simulink model "VIRTUAL_self_driving_stack_autoLocalize_v2"  (R2026a)
settings: Solver=ode1  StopTime=inf  FixedStep=1/500  EnableMultiTasking=on
values from neighbouring files (symbols this model uses):
  path_x4 = [-0.614 -0.604 -0.594 -0.584 -0.574 -0.564 -0.554 -0.544 -0.534 -0.524 -0.514 -0.504 ... (1761 elements, 1761x1)]    [SDCS_Paths_7.mat]
  path_y4 = [-1.0887 -1.0887 -1.0887 -1.0887 -1.0887 -1.0887 -1.0887 -1.0887 -1.0887 -1.0887 -1.0887 -1.0887 ... (1761 elements, 1761x1)]    [SDCS_Paths_7.mat]
undefined symbols (not defined in the file or in its folder): AAAF5050, CSI_Sample_Time, DiscIntNeverNeededParam, gcbh, height, HIL, ImageDisplay_Sample_Time, Initialization_Time, JPEG, K12, left, LiDAR_Sample_Time, MC, qc_get_step_size, RealSense_Sample_Time, top, video_display_show, width
libraries: quarc_library x67, simulink x5, visionconversions x1, visiontransforms x1, sl_discontinuities x1
(part 3 of 3)

== system VIRTUAL_self_driving_stack_autoLocalize_v2/rateTimingPlots/monitorTiming5 ==
  note: moniorTiming Module:
      |
      | This subsystem outputs the sample time and computation time of the model.
      |
      | Outputs:
      | sampleTime (s) n/a : Sample time (unfiltered and filtered) in seconds.
      | computationTime (s) n/a : Computation time (unfiltered and filtered) in seconds.
      |
      | Usage:
      | Compare the Sample Time (s) output to a constant (qc_get_step_size) to monitor whether or not the desired sample time is being achieved. The Computation Time (s) values should be lower than the corresponding sample time value to ensure that the solver has enough time per time step.
  note: Timing Performance
  Computation Time : quarc_library/Sources/Time/Computation Time  sample_time=LiDAR_Sample_Time  use_model=on  use_cpu_time=off
  Constant : Constant  Value=LiDAR_Sample_Time  SampleTime=-1
  Mux : Mux  Inputs=3
  Sample Time : quarc_library/Sources/Time/Sample Time  Priority=-99  sample_time=LiDAR_Sample_Time
  Timing (s) : Outport  VectorParamsAs1DForOutWhenUnconnected=off
  wires:
  Constant/1 -> Mux/2
  Sample Time/1 -> Mux/1
  Mux/1 -> Timing (s)/1
  Computation Time/1 -> Mux/3

== system VIRTUAL_self_driving_stack_autoLocalize_v2/rateTimingPlots/monitorTiming7 ==
  note: Timing Performance
  note: moniorTiming Module:
      |
      | This subsystem outputs the sample time and computation time of the model.
      |
      | Outputs:
      | sampleTime (s) n/a : Sample time (unfiltered and filtered) in seconds.
      | computationTime (s) n/a : Computation time (unfiltered and filtered) in seconds.
      |
      | Usage:
      | Compare the Sample Time (s) output to a constant (qc_get_step_size) to monitor whether or not the desired sample time is being achieved. The Computation Time (s) values should be lower than the corresponding sample time value to ensure that the solver has enough time per time step.
  Computation Time : quarc_library/Sources/Time/Computation Time  sample_time=1  use_model=on  use_cpu_time=off
  Constant : Constant  SampleTime=-1
  Mux : Mux  Inputs=3
  Sample Time : quarc_library/Sources/Time/Sample Time  Priority=-99  sample_time=1
  Timing (s) : Outport  VectorParamsAs1DForOutWhenUnconnected=off
  wires:
  Computation Time/1 -> Mux/3
  Mux/1 -> Timing (s)/1
  Sample Time/1 -> Mux/1
  Constant/1 -> Mux/2

== system VIRTUAL_self_driving_stack_autoLocalize_v2/readQCarDAC/counts to meters ==
  note: Estimate car speed from motor encoder counts rate
  note: v = 2*pi*r * omega (if omega is in rot/s)
      | v = r * omega (if omega is in rad/s)
      | r = 0.0342 m
  note: (Diff. pinion*pinion)/(Spur*Diff. spur)
  note: speedEstimation Module:
      |
      | This subsystem converts the motor speed measurements in counts/s to a useful longitudinal car speed in m/s.
      |
      | Inputs:
      | motorSpeed (counts/s) n/a : Drive motor speed measured using an encoder
      |
      | Outputs:
      | longitudinalCarSpeed (m/s) n/a : The platform's longitudinal speed (along the front-rear axis direction)
  motorSpeed (counts/s) : Inport
  counts to rotations : Gain  Gain=1/720/4
  gear ratios : Gain  Gain=(13*19)/(70*37)
  rot/s to rad/s : Gain  Gain=2*pi
  wheel radius : Gain  Gain=0.0342
  longitudinalCarSpeed (m/s) : Outport  VectorParamsAs1DForOutWhenUnconnected=off
  wires:
  motorSpeed (counts/s)/1 -> counts to rotations/1
  rot/s to rad/s/1 -> wheel radius/1  "wheel speed (rad/s)"
  counts to rotations/1 -> gear ratios/1  "motor speed (rot/s)"
  wheel radius/1 -> longitudinalCarSpeed (m/s)/1  "wheel speed (m/s)"
  gear ratios/1 -> rot/s to rad/s/1  "shaft speed (rots/s)"

== system VIRTUAL_self_driving_stack_autoLocalize_v2/readQCarDAC/counts//s to m//s ==
  note: speedEstimation Module:
      |
      | This subsystem converts the motor speed measurements in counts/s to a useful longitudinal car speed in m/s.
      |
      | Inputs:
      | motorSpeed (counts/s) n/a : Drive motor speed measured using an encoder
      |
      | Outputs:
      | longitudinalCarSpeed (m/s) n/a : The platform's longitudinal speed (along the front-rear axis direction)
  note: (Diff. pinion*pinion)/(Spur*Diff. spur)
  note: v = 2*pi*r * omega (if omega is in rot/s)
      | v = r * omega (if omega is in rad/s)
      | r = 0.0342 m
  note: Estimate car speed from motor encoder counts rate
  motorSpeed (counts/s) : Inport
  counts to rotations : Gain  Gain=1/720/4
  gear ratios : Gain  Gain=(13*19)/(70*37)
  rot/s to rad/s : Gain  Gain=2*pi
  wheel radius : Gain  Gain=0.0342
  longitudinalCarSpeed (m/s) : Outport  VectorParamsAs1DForOutWhenUnconnected=off
  wires:
  gear ratios/1 -> rot/s to rad/s/1  "shaft speed (rots/s)"
  wheel radius/1 -> longitudinalCarSpeed (m/s)/1  "wheel speed (m/s)"
  counts to rotations/1 -> gear ratios/1  "motor speed (rot/s)"
  rot/s to rad/s/1 -> wheel radius/1  "wheel speed (rad/s)"
  motorSpeed (counts/s)/1 -> counts to rotations/1

== system VIRTUAL_self_driving_stack_autoLocalize_v2/readQCarDAC/powerConsumptionMonitor ==
  note: Battery percentage calculation
  note: P = VI
  note: Electrical
      | power
      | consumed
  note: Power Monitoring Module:
      |
      | This subsystem monitors power consumption and provides a percentage battery remaining indicator.
      |
      | Inputs:
      | motorCurrent (A) n/a : Motor current being pulled by the main drive motor
      | batteryVoltage (V) {0, 12.6} : Current battery voltage reading
      |
      | Outputs:
      | motorPowerConsumption (W) n/a : Current power in Watts being pulled by the main drive motor
      | batteryLevel (%) {0,1} : Percentage battery level remaining
      |
      | Usage:
      | This is based on a maximum 3S battery voltage of 12.6 V (4.2V per cell) and minimum of 10.5 V (3.5V per cell)
  motorCurrent (A) [1] : Inport
  batteryVoltage (V) [1] : Inport  Port=2
  Divide : Product  Inputs=*/
  Gain : Gain  Gain=100
  Product : Product
  Subtract : Sum  Inputs=+-
  Subtract1 : Sum  Inputs=+-
  max voltage : Constant  Value=12.6
  min voltage : Constant  Value=10.5
  motorPowerConsumption (W) [1] : Outport  VectorParamsAs1DForOutWhenUnconnected=off
  batteryLevel (%) [1] : Outport  Port=2  VectorParamsAs1DForOutWhenUnconnected=off
  wires:
  Divide/1 -> Gain/1
  Subtract1/1 -> Divide/2
  Gain/1 -> batteryLevel (%) [1]/1
  Product/1 -> motorPowerConsumption (W) [1]/1
  min voltage/1 -> Subtract/2, Subtract1/2
  motorCurrent (A) [1]/1 -> Product/1
  max voltage/1 -> Subtract1/1
  Subtract/1 -> Divide/1
  batteryVoltage (V) [1]/1 -> Subtract/1, Product/2

== system VIRTUAL_self_driving_stack_autoLocalize_v2/speedController/realsenseObstacleDetectionSpeedAdjust ==
  obstacleDistance [1] (m) : Inport
  desiredSpeed [1] (m/s) : Inport  Port=2
  Constant : Constant  Value=0.375
  Constant2 : Constant  Value=0.6
  MATLAB Function : MATLAB Function  TreatAsAtomicUnit=on
  objectDetectionAdjustedSpeed [1] (m/s) : Outport  VectorParamsAs1DForOutWhenUnconnected=off
  wires:
  Constant2/1 -> MATLAB Function/3(nominal_tracking_distance)  "nominal tracking distance (m)"
  Constant/1 -> MATLAB Function/2(stop_distance)  "stop distance (m)"
  obstacleDistance [1] (m)/1 -> MATLAB Function/1(obstacle_distance)
  MATLAB Function/1(speed_cmd) -> objectDetectionAdjustedSpeed [1] (m/s)/1
  desiredSpeed [1] (m/s)/1 -> MATLAB Function/4(nominal_speed)

== system VIRTUAL_self_driving_stack_autoLocalize_v2/speedController/speedController ==
  note: Feedforward
  note: Feedback
  arm [1] (bool) : Inport
  desiredSpeed (m/s) : Inport  Port=2
  currentSpeed (m/s) : Inport  Port=3
  Add : Sum
  Add1 : Sum
  Compare To Zero : simulink/Logic and Bit Operations/Compare To Zero  relop===  OutDataTypeStr=boolean
  Integrator1 : Integrator  ExternalReset=either  LimitOutput=on  UpperSaturationLimit=0.4  LowerSaturationLimit=-0.4
  Kff (% / m/s) : Gain  Gain=0.1
  "Ki (% / m) " : Gain
  Kp (% / m/s) : Gain  Gain=.3
  Multiply : Product
  Multiply1 : Product
  Multiply2 : Product
  Speed_Tracking : Scope  NumInputPorts=2
  Sum : Sum  Inputs=|+-
  command saturation : Saturate  UpperLimit=5  LowerLimit=-5
  throttleCmd (%) : Outport  VectorParamsAs1DForOutWhenUnconnected=off
  wires:
  command saturation/1 -> Multiply1/1  "desired"
  arm [1] (bool)/1 -> Multiply2/2, Multiply1/2, Multiply/2
  currentSpeed (m/s)/1 -> Multiply/1  "meas"
  Multiply/1 -> Sum/2, Speed_Tracking/2  "measured"
  Add/1 -> Add1/2
  Add1/1 -> Multiply2/1  "%"
  Multiply1/1 -> Compare To Zero/1, Sum/1, Kff (% / m/s)/1, Speed_Tracking/1  "desired"
  Integrator1/1 -> Add/2
  Kp (% / m/s)/1 -> Add/1
  Compare To Zero/1 -> Integrator1/2
  Kff (% / m/s)/1 -> Add1/1
  Sum/1 -> "Ki (% / m) "/1, Kp (% / m/s)/1
  "Ki (% / m) "/1 -> Integrator1/1
  Multiply2/1 -> throttleCmd (%)/1  "pwm duty cycle"
  desiredSpeed (m/s)/1 -> command saturation/1

== system VIRTUAL_self_driving_stack_autoLocalize_v2/speedController/stopSignDetectionSpeedAdjust ==
  stopSignDetection : Inport
  speedIn : Inport  Port=2
  Constant : Constant  Value=0
  Display : Display
  Display1 : Display
  Elapsed : Scope
      settings: ActiveDisplayYMinimum=-1  ActiveDisplayYMaximum=1
  Less Than Threshold : Subsystem
  NOT : Logic  Operator=NOT  IconShape=distinctive  AllPortsSameDT=off  OutDataTypeStr=boolean
  OR : Logic  Operator=OR  IconShape=distinctive  AllPortsSameDT=off  OutDataTypeStr=boolean
  Switch : Switch  Criteria=u2 > Threshold  SaturateOnIntegerOverflow=off  InputSameDT=off
  Switch1 : Switch  Criteria=u2 > Threshold  SaturateOnIntegerOverflow=off  InputSameDT=off
  time elspsed or no stop sign : Display
  time within stop sign : Constant  Value=2
  speedOut : Outport  VectorParamsAs1DForOutWhenUnconnected=off
  wires:
  stopSignDetection/1 -> NOT/1, Display1/1, Switch/2, Less Than Threshold/1(signal)
  time within stop sign/1 -> Less Than Threshold/2(Duration Threshold)
  Constant/1 -> Switch/1
  speedIn/1 -> Switch1/1, Switch/3
  Less Than Threshold/1(elapsed) -> OR/2, Elapsed/1
  NOT/1 -> OR/1
  OR/1 -> Switch1/2, time elspsed or no stop sign/1
  Switch/1 -> Switch1/3
  Switch1/1 -> Display/1, speedOut/1

== system VIRTUAL_self_driving_stack_autoLocalize_v2/speedController/turnSpeedHandler ==
  speedCmd [1] (m/s) : Inport
  steeringCmd [1] (rad) : Inport  Port=2
  Cos ^ (attentuation) : Inport  Port=3
  Cos : Trigonometry  Operator=cos
  Product : Product
  Speed Comparison : Scope  NumInputPorts=2
  Square : Math  Operator=pow  SignedPower=on
  attenuationLimits : Saturate  UpperLimit=1  LowerLimit=.3
  attenuatedSpeedCmd [1] (m/s) : Outport  VectorParamsAs1DForOutWhenUnconnected=off
  wires:
  Cos/1 -> Square/1
  attenuationLimits/1 -> Product/2
  speedCmd [1] (m/s)/1 -> Product/1, Speed Comparison/1  "Input Speed"
  Cos ^ (attentuation)/1 -> Square/2
  Square/1 -> attenuationLimits/1
  Product/1 -> attenuatedSpeedCmd [1] (m/s)/1, Speed Comparison/2
  steeringCmd [1] (rad)/1 -> Cos/1  "input steering"

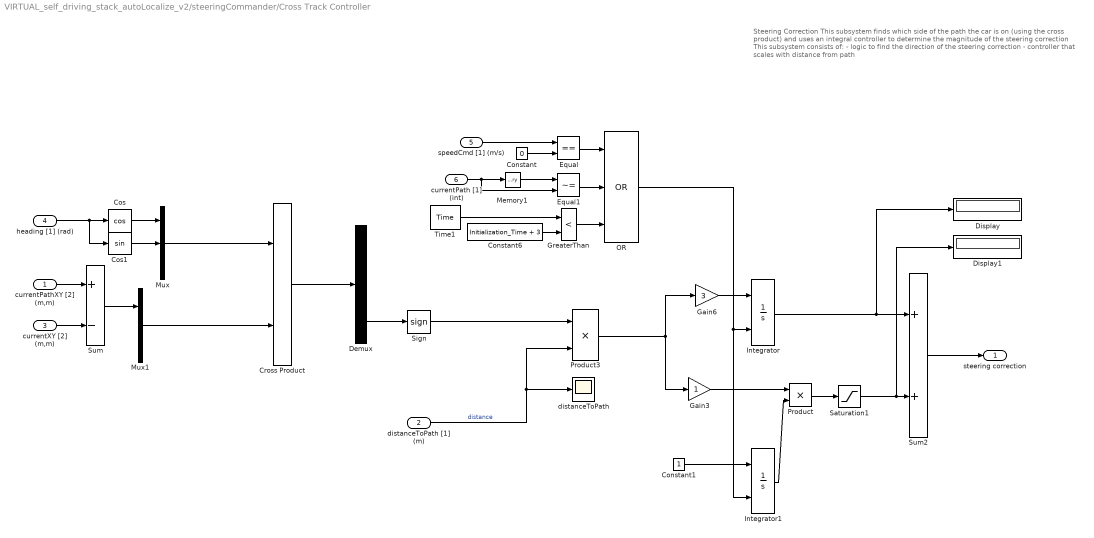
== system VIRTUAL_self_driving_stack_autoLocalize_v2/steeringCommander/Cross Track Controller ==
  note: Steering Correction
      |
      | This subsystem finds which side of the path the car is on (using the cross product) and uses an integral controller to determine the magnitude of the steering correction
      |
      | This subsystem consists of:
      |
      | - logic to find the direction of the steering correction
      | - controller that scales with distance from path
  currentPathXY [2] (m,m) : Inport
  distanceToPath [1] (m) : Inport  Port=2
  currentXY [2] (m,m) : Inport  Port=3
  heading [1] (rad) : Inport  Port=4
  speedCmd [1] (m/s) : Inport  Port=5
  currentPath [1] (int) : Inport  Port=6
  Constant : Constant  Value=0
  Constant1 : Constant
  Constant6 : Constant  Value=Initialization_Time + 3
  Cos : Trigonometry  Operator=cos
  Cos1 : Trigonometry
  Cross Product : quarc_library/Math Operations/Vectors/Cross Product
      settings: SourceProductName=QUARC Targets
  Demux : Demux  Outputs=3
  Display : Display
  Display1 : Display
  Equal : RelationalOperator  Operator===  OutDataTypeStr=boolean  RndMeth=Simplest  InputSameDT=off
  Equal1 : RelationalOperator  Operator=~=  OutDataTypeStr=boolean  RndMeth=Simplest  InputSameDT=off
  Gain3 : Gain
  Gain6 : Gain  Gain=3
  GreaterThan : RelationalOperator  Operator=<  OutDataTypeStr=boolean  RndMeth=Simplest  InputSameDT=off
  Integrator : Integrator  ExternalReset=level  LimitOutput=on  UpperSaturationLimit=.2  LowerSaturationLimit=-.2
  Integrator1 : Integrator  ExternalReset=level  LimitOutput=on  UpperSaturationLimit=1  LowerSaturationLimit=0
  Memory1 : Memory  InitialCondition=6  InheritSampleTime=on  LinearizeMemory=on  LinearizeAsDelay=on
  Mux : Mux  Inputs=3
  Mux1 : Mux  Inputs=2
  OR : Logic  Operator=OR  Inputs=3  IconShape=distinctive  AllPortsSameDT=off  OutDataTypeStr=boolean
  Product : Product
  Product3 : Product
  Saturation1 : Saturate  UpperLimit=.2  LowerLimit=-.2
  Sign : Signum
  Sum : Sum  Inputs=+-
  Sum2 : Sum
  Time1 : quarc_library/Sources/Time/Time  time_source=Wall clock  sample_time=qc_get_step_size
  distanceToPath : Scope
  steering correction : Outport
  wires:
  heading [1] (rad)/1 -> Cos1/1, Cos/1
  Cos/1 -> Mux/1
  Cos1/1 -> Mux/2
  currentXY [2] (m,m)/1 -> Sum/2
  currentPathXY [2] (m,m)/1 -> Sum/1
  Sum/1 -> Mux1/1
  Mux1/1 -> Cross Product/2
  Mux/1 -> Cross Product/1
  Cross Product/1 -> Demux/1
  Demux/3 -> Sign/1
  Sign/1 -> Product3/1
  Gain6/1 -> Integrator/1
  Product3/1 -> Gain3/1, Gain6/1
  Integrator/1 -> Display/1, Sum2/1
  Saturation1/1 -> Display1/1, Sum2/2
  distanceToPath [1] (m)/1 -> Product3/2, distanceToPath/1  "distance"
  Sum2/1 -> steering correction/1
  speedCmd [1] (m/s)/1 -> Equal/1
  Constant/1 -> Equal/2
  currentPath [1] (int)/1 -> Equal1/2, Memory1/1
  Memory1/1 -> Equal1/1
  Equal1/1 -> OR/2
  Equal/1 -> OR/1
  OR/1 -> Integrator1/2, Integrator/2
  Constant1/1 -> Integrator1/1
  Product/1 -> Saturation1/1
  Gain3/1 -> Product/1
  Integrator1/1 -> Product/2
  Time1/1 -> GreaterThan/1
  Constant6/1 -> GreaterThan/2
  GreaterThan/1 -> OR/3

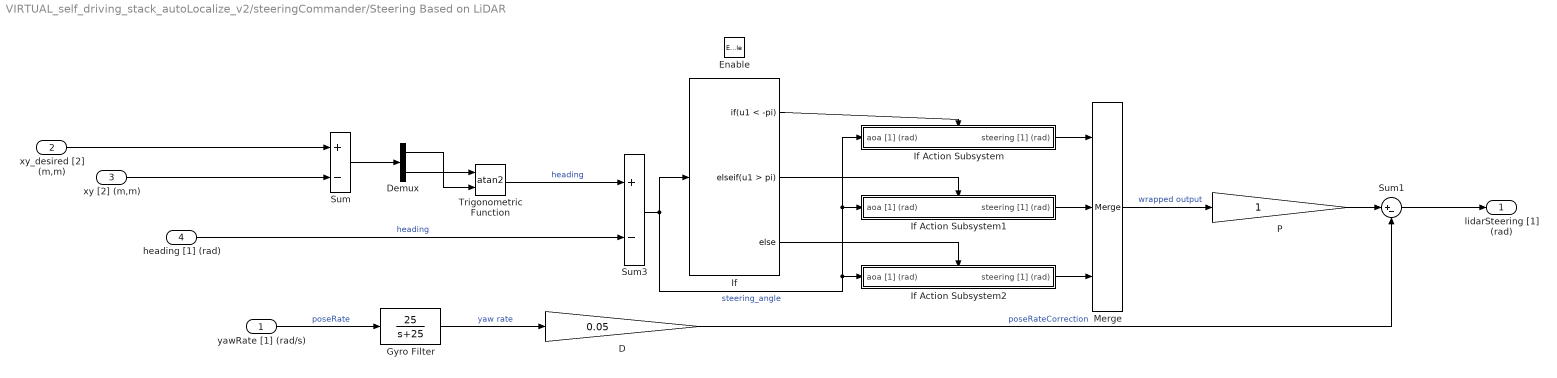
== system VIRTUAL_self_driving_stack_autoLocalize_v2/steeringCommander/Steering Based on LiDAR ==
  yawRate [1] (rad/s) : Inport
  xy_desired [2] (m,m) : Inport  Port=2
  xy [2] (m,m) : Inport  Port=3
  heading [1] (rad) : Inport  Port=4
  Enable : EnablePort  PropagateVarSize=During execution
  D : Gain  Gain=0.05
  Demux : Demux  Outputs=2
  Gyro Filter : TransferFcn  Numerator=[25]  Denominator=[1 25]
  If : If  IfExpression=u1 < -pi  ElseIfExpressions=u1 > pi
  If Action Subsystem : Subsystem  TreatAsAtomicUnit=on
  If Action Subsystem1 : Subsystem  TreatAsAtomicUnit=on
  If Action Subsystem2 : Subsystem  TreatAsAtomicUnit=on
  Merge : Merge  Inputs=3
  P : Gain
  Sum : Sum  Inputs=+-
  Sum1 : Sum  Inputs=|+-
  Sum3 : Sum  Inputs=+-
  Trigonometric Function : Trigonometry  Operator=atan2
  lidarSteering [1] (rad) : Outport
  wires:
  If/1 -> If Action Subsystem/Action
  If/2 -> If Action Subsystem1/Action
  If/3 -> If Action Subsystem2/Action
  Sum3/1 -> If Action Subsystem1/1(aoa [1] (rad)), If Action Subsystem/1(aoa [1] (rad)), If Action Subsystem2/1(aoa [1] (rad)), If/1  "steering_angle"
  If Action Subsystem/1(steering [1] (rad)) -> Merge/1
  If Action Subsystem1/1(steering [1] (rad)) -> Merge/2
  If Action Subsystem2/1(steering [1] (rad)) -> Merge/3
  Demux/1 -> Trigonometric Function/2
  xy [2] (m,m)/1 -> Sum/2
  xy_desired [2] (m,m)/1 -> Sum/1
  heading [1] (rad)/1 -> Sum3/2  "heading"
  Sum/1 -> Demux/1
  Demux/2 -> Trigonometric Function/1
  Merge/1 -> P/1  "wrapped output"
  D/1 -> Sum1/2  "poseRateCorrection"
  Sum1/1 -> lidarSteering [1] (rad)/1
  P/1 -> Sum1/1
  Trigonometric Function/1 -> Sum3/1  "heading"
  yawRate [1] (rad/s)/1 -> Gyro Filter/1  "poseRate"
  Gyro Filter/1 -> D/1  "yaw rate"

== system VIRTUAL_self_driving_stack_autoLocalize_v2/HSVStopSignDetection/findStopSignDistance/Depth Image (m) ==
  In1 : Inport
  Channel : quarc_library/Signal Routing/Channel  channel=0  buffer_size=1
  Image Compress : quarc_library/Image Processing/Generic/Image Compress  algorithm=JPEG  source=Internal dialog parameter  quality=quality  output_dim=-1
  Video Display : quarc_library/Multimedia/Video Display  Tag=VIRTUAL_self_driving_stack_autoLocalize_v2/HSVStopSignDetection/findStopSignDistance/Depth Image (m)/Video Display  sample_time=sample_time  use_hardware=on
  wires:
  Image Compress/1 -> Channel/1
  In1/1 -> Image Compress/1
  Channel/1 -> Video Display/1

== system VIRTUAL_self_driving_stack_autoLocalize_v2/HSVStopSignDetection/findStopSignLocation/Binary showing blob found ==
  In1 : Inport
  Channel : quarc_library/Signal Routing/Channel  channel=1  buffer_size=1
  Image Compress : quarc_library/Image Processing/Generic/Image Compress  algorithm=JPEG  source=Internal dialog parameter  quality=quality  output_dim=-1
  Video Display : quarc_library/Multimedia/Video Display  Tag=<binary blob, 124 chars, not shown>  sample_time=sample_time  use_hardware=on
  wires:
  Image Compress/1 -> Channel/1
  In1/1 -> Image Compress/1
  Channel/1 -> Video Display/1

== system VIRTUAL_self_driving_stack_autoLocalize_v2/HSVStopSignDetection/findStopSignLocation/Raw RGB ==
  In1 : Inport
  Channel : quarc_library/Signal Routing/Channel  channel=2  buffer_size=1
  Image Compress : quarc_library/Image Processing/Generic/Image Compress  algorithm=JPEG  source=Internal dialog parameter  quality=quality  output_dim=-1
  Video Display : quarc_library/Multimedia/Video Display  Tag=VIRTUAL_self_driving_stack_autoLocalize_v2/HSVStopSignDetection/findStopSignLocation/Raw RGB/Video Display  sample_time=sample_time  use_hardware=on
  wires:
  Image Compress/1 -> Channel/1
  In1/1 -> Image Compress/1
  Channel/1 -> Video Display/1

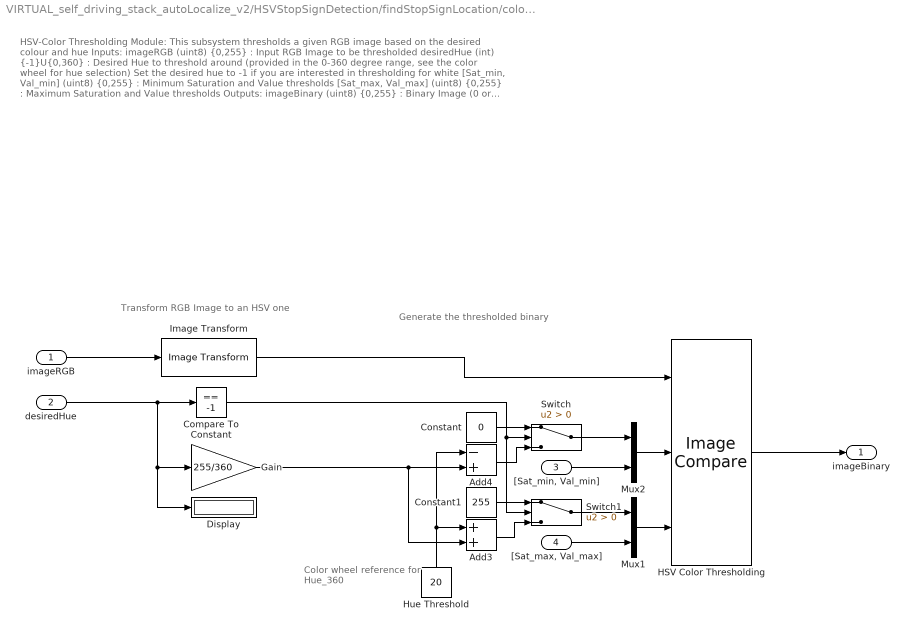
== system VIRTUAL_self_driving_stack_autoLocalize_v2/HSVStopSignDetection/findStopSignLocation/colorThresholdingHSV ==
  note: Generate the thresholded binary
  note: Transform RGB Image to an HSV one
  note: Color wheel
      | reference
      | for Hue_360
  note: HSV-Color Thresholding Module:
      |
      | This subsystem thresholds a given RGB image based on the desired colour and hue
      |
      | Inputs:
      | imageRGB (uint8) {0,255} : Input RGB Image to be thresholded
      | desiredHue (int) {-1}U{0,360} : Desired Hue to threshold around (provided in the 0-360 degree range, see the color wheel for hue selection)
      | Set the desired hue to -1 if you are interested in thresholding for white
      | [Sat_min, Val_min] (uint8) {0,255} : Minimum Saturation and Value thresholds
      | [Sat_max, Val_max] (uint8) {0,255} : Maximum Saturation and Value thresholds
      |
      | Outputs:
      | imageBinary (uint8) {0,255} : Binary Image (0 or 255 and no other value) representing the thresholding output
      |
      | Usage:
      | This module can be used when you are interested in thresholding for a certain hue regardless of the luminance. Compared to RGB thresholding which does not work well when the lighting conditions vary, HSV thresholding will correctly threshold for a hue (color) and allow you to specify a broad range of illuminance via the saturation and value thresholds. To broaden the range of hues accepted in the thresholding block, increase the Hue Threshold parameter.
  imageRGB : Inport
  desiredHue : Inport  Port=2
  "[Sat_min, Val_min]" : Inport  Port=3
  "[Sat_max, Val_max]" : Inport  Port=4
  Add3 : Sum
  Add4 : Sum  Inputs=-+
  Compare To Constant : simulink/Logic and Bit Operations/Compare To Constant  relop===  const=-1  OutDataTypeStr=boolean
  Constant : Constant  Value=0
  Constant1 : Constant  Value=255
  Display : Display
  Gain : Gain  Gain=255/360
  HSV Color Thresholding : quarc_library/Image Processing/Generic/Image Compare  output_type=Combined (one HxW output)  source=External input ports  r_comparison=min <= pixel and pixel <= max with wrapping  r_minimum=30  r_maximum=70  g_comparison=min <= pixel and pixel <= max  g_minimum=60  g_maximum=100  b_comparison=min <= pixel and pixel <= max  b_minimum=40  b_maximum=80
      settings: SourceProductName=QUARC Targets
  Hue Threshold : Constant  Value=20
  Image Transform : quarc_library/Image Processing/Generic/Image Transform  algorithm=RGB to HSV  color_theme=KRYGCBMW  min_pixel=0  max_pixel=4000  contour_depth=1  focal_length=308  principal_point=[262 334]  radial_coeffs=[-0.3129 0.0907]  tangential_coeffs=[]  extrapolated_pixel=0  interpolation=nearest  row_coords=0  column_coords=0  output_height=480  output_width=640  angle=0  origin=[240 320]  output_origin=[240 320]  output_data_type=uint8
      settings: AttributesFormatString=(%<algorithm>)  SourceProductName=QUARC Targets
  Mux1 : Mux  Inputs=2
  Mux2 : Mux  Inputs=2
  Switch : Switch  Criteria=u2 > Threshold  SaturateOnIntegerOverflow=off  InputSameDT=off
  Switch1 : Switch  Criteria=u2 > Threshold  SaturateOnIntegerOverflow=off  InputSameDT=off
  imageBinary : Outport  VectorParamsAs1DForOutWhenUnconnected=off
  wires:
  imageRGB/1 -> Image Transform/1
  Hue Threshold/1 -> Add3/1, Add4/1
  Image Transform/1 -> HSV Color Thresholding/1
  desiredHue/1 -> Compare To Constant/1, Display/1, Gain/1
  Gain/1 -> Add4/2, Add3/2
  Constant1/1 -> Switch1/1
  "[Sat_max, Val_max]"/1 -> Mux1/2
  Add3/1 -> Switch1/3
  Switch/1 -> Mux2/1
  Compare To Constant/1 -> Switch/2, Switch1/2
  Constant/1 -> Switch/1
  Switch1/1 -> Mux1/1
  Mux1/1 -> HSV Color Thresholding/3
  Add4/1 -> Switch/3
  "[Sat_min, Val_min]"/1 -> Mux2/2
  Mux2/1 -> HSV Color Thresholding/2
  HSV Color Thresholding/1 -> imageBinary/1

== system VIRTUAL_self_driving_stack_autoLocalize_v2/speedController/stopSignDetectionSpeedAdjust/Less Than Threshold ==
  note: Calculate Duration stop sign is in range
  signal : Inport
  Duration Threshold : Inport  Port=2
  Constant : Constant  Value=0
  Data Type Conversion : DataTypeConversion  SaturateOnIntegerOverflow=off  RndMeth=Floor
  Discrete-Time Integrator : DiscreteIntegrator  Priority=1  ExternalReset=level  SampleTime=qc_get_step_size  ICPrevOutput=DiscIntNeverNeededParam  ICPrevScaledInput=DiscIntNeverNeededParam
  Relational Operator : RelationalOperator  Operator=>  InputSameDT=off
  Relational Operator1 : RelationalOperator  InputSameDT=off
  Reset Condition : Logic  Operator=NOT  AllPortsSameDT=off  OutDataTypeStr=boolean
  elapsed : Outport  VectorParamsAs1DForOutWhenUnconnected=off
  wires:
  Data Type Conversion/1 -> Discrete-Time Integrator/1
  signal/1 -> Relational Operator/1
  Constant/1 -> Relational Operator/2
  Relational Operator/1 -> Data Type Conversion/1, Reset Condition/1
  Reset Condition/1 -> Discrete-Time Integrator/2
  Discrete-Time Integrator/1 -> Relational Operator1/1
  Duration Threshold/1 -> Relational Operator1/2
  Relational Operator1/1 -> elapsed/1

== system VIRTUAL_self_driving_stack_autoLocalize_v2/steeringCommander/Steering Based on LiDAR/If Action Subsystem ==
  aoa [1] (rad) : Inport
  Action Port : ActionPort  ActionPortLabel=if(u1 < -pi)
  Bias : Bias  Bias=2*pi  SaturateOnIntegerOverflow=off
  steering [1] (rad) : Outport
  wires:
  aoa [1] (rad)/1 -> Bias/1
  Bias/1 -> steering [1] (rad)/1

== system VIRTUAL_self_driving_stack_autoLocalize_v2/steeringCommander/Steering Based on LiDAR/If Action Subsystem1 ==
  aoa [1] (rad) : Inport
  Action Port : ActionPort  ActionPortLabel=elseif(u1 > pi)
  Bias : Bias  Bias=-2*pi  SaturateOnIntegerOverflow=off
  steering [1] (rad) : Outport
  wires:
  Bias/1 -> steering [1] (rad)/1
  aoa [1] (rad)/1 -> Bias/1

== system VIRTUAL_self_driving_stack_autoLocalize_v2/steeringCommander/Steering Based on LiDAR/If Action Subsystem2 ==
  aoa [1] (rad) : Inport
  Action Port : ActionPort  ActionPortLabel=else
  Bias : Bias  SaturateOnIntegerOverflow=off
  steering [1] (rad) : Outport
  wires:
  aoa [1] (rad)/1 -> Bias/1
  Bias/1 -> steering [1] (rad)/1

== matlab function VIRTUAL_self_driving_stack_autoLocalize_v2/pathPlanner/Path 4  Look Ahead Generator/Windowed Closest Point Locator *Feedback the location1 ==
  data: x input; location output; y input; x_array input; y_array input; window input; global_search input; distance output; previous_location input
function [location,distance] = find_closest_window_point(x,y,x_array,y_array, window, global_search, previous_location)
distance = 1e6;
location = previous_location;
array_length = length (x_array);

if (global_search == 1)
    
    %Search the whole array (usually at startup)
    for i =1:array_length
        d = (x-x_array(i))^2 + (y-y_array(i))^2;
        if d < distance
            distance = d;
            location = i;
        end
    end
    
else
    
    if (location + window) > array_length
        %We need to wrap from the end
        % loop one - end of array:
        for i = (location-window):array_length
            d = (x-x_array(i))^2 + (y-y_array(i))^2;
            if d < distance
                distance = d;
                location = i;
            end
        end
        % loop two - start of array:
        for i = 1:(location+window-array_length)
            d = (x-x_array(i))^2 + (y-y_array(i))^2;
            if d < distance
                distance = d;
                location = i;
            end
        end
        
    elseif (location-window) < 1
        %We need to wrap from the beginning
        % loop one - end of array:
        for i = (array_length+location-window):array_length
            d = (x-x_array(i))^2 + (y-y_array(i))^2;
            if d < distance
                distance = d;
                location = i;
            end
        end
        % loop two - start of array:
        for i = 1:(location+window)
            d = (x-x_array(i))^2 + (y-y_array(i))^2;
            if d < distance
                distance = d;
                location = i;
            end
        end
        
    else
        %no need to wrap
        for i = (location-window):(location+window)
            d = (x-x_array(i))^2 + (y-y_array(i))^2;
            if d < distance
                distance = d;
                location = i;
            end
        end
    end
    
end
distance = sqrt(distance);
end

== matlab function VIRTUAL_self_driving_stack_autoLocalize_v2/speedController/realsenseObstacleDetectionSpeedAdjust/MATLAB Function ==
  data: obstacle_distance input; speed_cmd output; stop_distance input; nominal_tracking_distance input; nominal_speed input
function speed_cmd = adaptive_cruise_control(obstacle_distance, stop_distance, nominal_tracking_distance, nominal_speed)

speed_cmd = nominal_speed;

if obstacle_distance < stop_distance
    speed_cmd = sat(nominal_speed,0,-1);
    
elseif obstacle_distance < nominal_tracking_distance
    speed_cmd = nominal_speed/(nominal_tracking_distance-stop_distance)*obstacle_distance...
        - nominal_speed/(nominal_tracking_distance-stop_distance)*stop_distance;
    
end

function output = sat (input, max,min)
if input > max
    output = max;
elseif input < min
    output = min;
else
    output = input;
end

== matlab function VIRTUAL_self_driving_stack_autoLocalize_v2/obstacleDetection/obstacleDetection Markham March 22/Draw Lines Module ==
  data: img_in input; img_out output; pts input; color input
function img_out = drawLines(img_in, pts, color)

% Draw lines connecting the points using the provided color

% Inputs:
% u         : Input RGB Image (size = m by n)
% pts       : p x-y pairs of points (px) where markers are to be drawn
% color     : 1x3 matrix of RGB color values for each marker

% Outputs:
% y         : Output RGB Image with the markers drawn in (size = m by n)

%% Initialization
if size(img_in, 3) == 3
    img_out = img_in;
elseif size(img_in, 3) == 1
    img_out = cat(3, img_in, img_in, img_in);
end

[p, ~] = size(pts); % determine the number of points

%% Draw the lines
    for i = 1:p-1
        % determine the max(rows_difference, col_difference) between two
        % points
        itr = max(abs(pts(i,1) - pts(i+1,1)), abs(pts(i,2) - pts(i+1,2)));
        
        % generate linear spaces of row and col values between the pts
        row_vec = round(linspace(pts(i,1), pts(i+1,1), itr));
        col_vec = round(linspace(pts(i,2), pts(i+1,2), itr));
        
        % iterate through the values and shade them right

        for j = 1:itr
            img_out(row_vec(j), col_vec(j),1) = color(1);
            img_out(row_vec(j), col_vec(j),2) = color(2);
            img_out(row_vec(j), col_vec(j),3) = color(3);
        end
    end
end

== matlab function VIRTUAL_self_driving_stack_autoLocalize_v2/obstacleDetection/obstacleDetection Markham March 22/Steering based image subselector ==
  data: pts output; depth input; distance output; steering input; minDistance input; maxDistance input; width input; height input; vertCenter input; maxSteering input; reduction input; maxSteeringWidth input
function [pts, distance] = estimateDepthInRegion(depth, steering, minDistance, maxDistance, width, height, vertCenter, maxSteering, reduction, maxSteeringWidth)
% Input: 640 x 360
[ROW, COL] = size(depth);
mark = COL/2 - (steering*(COL/2 - width/2)/maxSteering);
applied_width = max(width - abs(steering/maxSteeringWidth)*reduction*width, 60);
left_w = int32(max(mark+1-(applied_width/2), 0)); % pick the left end, but never let it get negative
right_w = int32(min(left_w + applied_width, COL)); % pick the right end, but never past the image width
upper_h = int32(max(ROW*vertCenter-height/2+1, 0)); % pick the upper end, but never let it get negative
lower_h = int32(min(ROW*vertCenter+height/2, ROW)); % pick the lower end, but never let it go past the image height
depth(:,1:40) = maxDistance; %this is to remove artifacts in the camera's left section
region = double(depth(upper_h:lower_h, left_w:right_w)); 
pts = double([upper_h, left_w; upper_h, right_w; lower_h, right_w; lower_h, left_w; upper_h, left_w]);
u_flat = reshape(region, 1, []);

temp = maxDistance*ones(1, length(u_flat));

for i = 1:length(u_flat)
    if (u_flat(i) >= minDistance) && (u_flat(i) <= maxDistance)
        temp(i) = u_flat(i);
    end
end

% u_flat(u_flat < minDistance) = [];
% u_flat(u_flat > maxDistance) = [];
% distance = mean(mean(u_flat));
distance = min(temp(:));
